simulink model "Debounce_Logic"  (R2024b)
settings: Solver=FixedStepDiscrete  StartTime=0.0  StopTime=10.0  FixedStep=0.001  MaxStep=0.001  RelTol=1e-3
undefined symbols (not defined in the file): TargetTime
settings Model: DataDictionary=DebounceLogic.sldd  Creator=User  LastModifiedBy=User

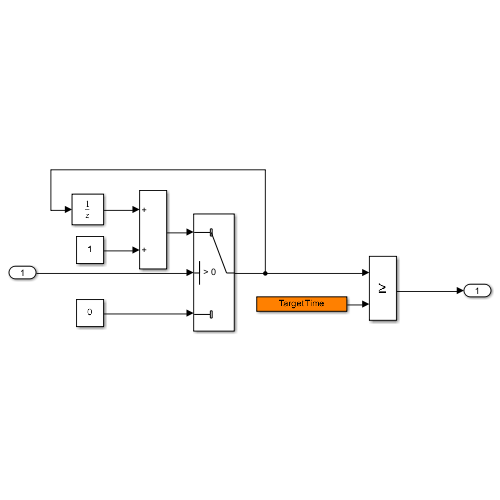
[thumbnail: Simulink's stored preview of the top-level diagram]
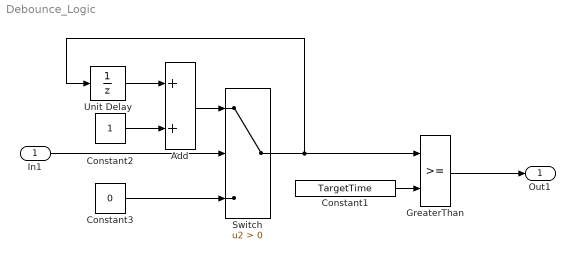
== system Debounce_Logic ==
  In1 : Inport  OutDataTypeStr=boolean
  Add : Sum
  Constant1 : Constant  Value=TargetTime
  Constant2 : Constant
  Constant3 : Constant  Value=0
  GreaterThan : RelationalOperator  OutDataTypeStr=boolean  RndMeth=Simplest  InputSameDT=off
  Switch : Switch  Criteria=u2 > Threshold  SaturateOnIntegerOverflow=off  InputSameDT=off
  Unit Delay : UnitDelay  SampleTime=-1  HasFrameUpgradeWarning=on
  Out1 : Outport
  wires:
  Add/1 -> Switch/1
  Unit Delay/1 -> Add/1
  Switch/1 -> Unit Delay/1, GreaterThan/1
  Constant1/1 -> GreaterThan/2
  Constant2/1 -> Add/2
  Constant3/1 -> Switch/3
  In1/1 -> Switch/2
  GreaterThan/1 -> Out1/1
